simulink model "Model_31_02_4"  (R2024b)
settings: Solver=FixedStepAuto  StartTime=0.0  StopTime=5  FixedStep=0.001  RelTol=1e-3
values from neighbouring files (symbols this model uses):
  g = pend1.g    [InversePODE.m]    (also in Laboratorio_2_Pendolo_inverso.m = 9.81; Laboratorio_2_Pendolo_inverso_conflict_copy_PC_2025_04_15.m = 9.81; Laboratorio_2_Pendolo_inverso_struct.m; TESTTT.m = 9.81)
  Kd = 2*psi*wn / a    (= 7.44876)    [Laboratorio_2_Pendolo_inverso_conflict_copy_PC_2025_04_15.m]    (also in Laboratorio_2_Pendolo_inverso_struct.m; TESTTT.m)
  Kp = (wn^2+b) /a    (= 60.059025)    [Laboratorio_2_Pendolo_inverso_conflict_copy_PC_2025_04_15.m]    (also in Laboratorio_2_Pendolo_inverso_struct.m; TESTTT.m)
  l = pend1.l    [InversePODE.m]    (also in Laboratorio_2_Pendolo_inverso.m = 0.75; Laboratorio_2_Pendolo_inverso_conflict_copy_PC_2025_04_15.m = 0.75; Laboratorio_2_Pendolo_inverso_struct.m; TESTTT.m = 0.75)
  M = pend1.M    [InversePODE.m]    (also in Laboratorio_2_Pendolo_inverso.m = 3; Laboratorio_2_Pendolo_inverso_conflict_copy_PC_2025_04_15.m = 3; Laboratorio_2_Pendolo_inverso_struct.m; TESTTT.m = 3)
  m = pend1.m    [InversePODE.m]    (also in Laboratorio_2_Pendolo_inverso.m = 0.1; Laboratorio_2_Pendolo_inverso_conflict_copy_PC_2025_04_15.m = 0.1; Laboratorio_2_Pendolo_inverso_struct.m; TESTTT.m = 0.1)
  x02 = [0;0;0;0]    [Laboratorio_2_Pendolo_inverso.m]    (also in Laboratorio_2_Pendolo_inverso_conflict_copy_PC_2025_04_15.m; Laboratorio_2_Pendolo_inverso_struct.m; TESTTT.m)
settings Model: Creator=baron  LastModifiedBy=baron

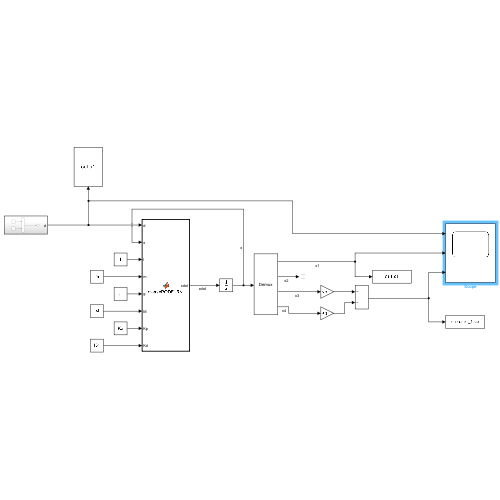
[thumbnail: Simulink's stored preview of the top-level diagram]
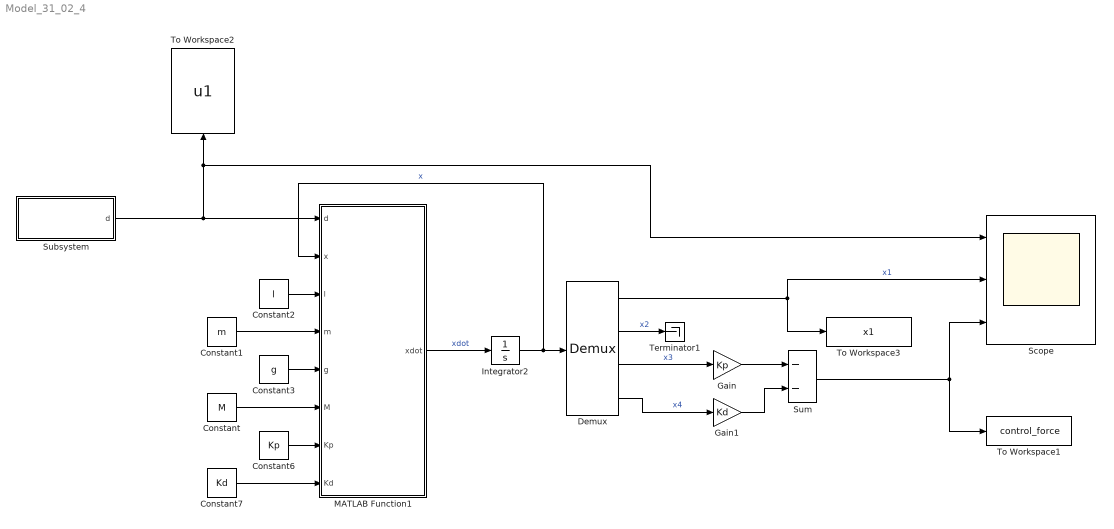
== system Model_31_02_4 ==
  Constant : Constant  Value=M
  Constant1 : Constant  Value=m
  Constant2 : Constant  Value=l
  Constant3 : Constant  Value=g
  Constant6 : Constant  Value=Kp
  Constant7 : Constant  Value=Kd
  Demux : Demux
      settings: DisplayOption=none
  Gain : Gain  Gain=Kp
  Gain1 : Gain  Gain=Kd
  Integrator2 : Integrator  InitialCondition=x02
  MATLAB Function1 : MATLAB Function  TreatAsAtomicUnit=on
  Scope : Scope  NumInputPorts=3
  Subsystem : Subsystem
  Sum : Sum  Inputs=--
  Terminator1 : Terminator
  To Workspace1 : ToWorkspace  VariableName=control_force  SampleTime=-1
      settings: Save2DSignal=2-D array (concatenate along first dimension)
  To Workspace2 : ToWorkspace  VariableName=u1  SampleTime=-1
      settings: Save2DSignal=2-D array (concatenate along first dimension)
  To Workspace3 : ToWorkspace  VariableName=x1  SampleTime=-1
      settings: Save2DSignal=2-D array (concatenate along first dimension)
  wires:
  Constant1/1 -> MATLAB Function1/4(m)
  Constant3/1 -> MATLAB Function1/5(g)
  Constant/1 -> MATLAB Function1/6(M)
  Integrator2/1 -> MATLAB Function1/2(x), Demux/1  "x"
  Constant2/1 -> MATLAB Function1/3(l)
  Sum/1 -> Scope/3, To Workspace1/1
  MATLAB Function1/1(xdot) -> Integrator2/1  "xdot"
  Demux/1 -> To Workspace3/1, Scope/2  "x1"
  Subsystem/1(d) -> Scope/1, To Workspace2/1, MATLAB Function1/1(d)
  Constant6/1 -> MATLAB Function1/7(Kp)
  Constant7/1 -> MATLAB Function1/8(Kd)
  Demux/3 -> Gain/1  "x3"
  Gain/1 -> Sum/1
  Gain1/1 -> Sum/2
  Demux/2 -> Terminator1/1  "x2"
  Demux/4 -> Gain1/1  "x4"

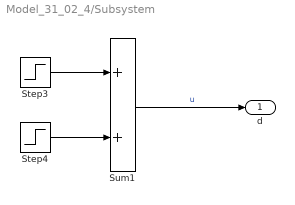
== system Model_31_02_4/Subsystem ==
  Step3 : Step  Time=0  SampleTime=0
  Step4 : Step  Time=.1  After=-1  SampleTime=0
  Sum1 : Sum
  d : Outport
  wires:
  Sum1/1 -> d/1  "u"
  Step4/1 -> Sum1/2
  Step3/1 -> Sum1/1

== matlab function Model_31_02_4/MATLAB Function1 ==
  data: d input; xdot output; x input; l input; m input; g input; M input; Kp input; Kd input
function xdot = InversePODE_RNL(d,x,l,m,g,M,Kp,Kd)
    x1 = x(1);
    x2 = x(2);
    x3 = x(3);
    x4 = x(4);
    

    xdot1 = x2;
    xdot2 = (+ m*g*sin(x3)*cos(x3) - m*l*(x4^2)*sin(x3)  + ((-Kp*x3-Kd*x4) + d))/(M+m-(m*cos(x3)^2));
    xdot3 = x4;
    xdot4 = ((-m)/(M+m)*(x4^2)*cos(x3)*sin(x3)  + ((-Kp*x3-Kd*x4) + d)/((M+m)*l)*cos(x3) +g/l*sin(x3))/(1-m/(M+m)*(cos(x3)^2));


    xdot= [xdot1; xdot2; xdot3; xdot4];
end
